simulink model "IRB120_identification"  (R2026a)
settings: Solver=ode3  StopTime=40  FixedStep=0.004
InitFcn:
  | addpath(fullfile(fileparts(get_param(bdroot, 'FileName')), 'meshes'));
values from neighbouring files (symbols this model uses):
  m = b.Mass    [extract_nominal_parameters.m]
  N = size(m.q, 1)    [build_and_simulate.m]
  s = min(t/cfg.T_ramp, 1)    [build_and_simulate.m]
  X = Tm \ getTransform(r, qm, bodies{i})    [extract_nominal_parameters.m]
undefined symbols (not defined in the file or in its folder): Y, Z
libraries: sm_lib x62, nesl_utility x31
(part 1 of 2)
settings Model: Creator=Muhammad Adel  LastModifiedBy=Muhammad Adel

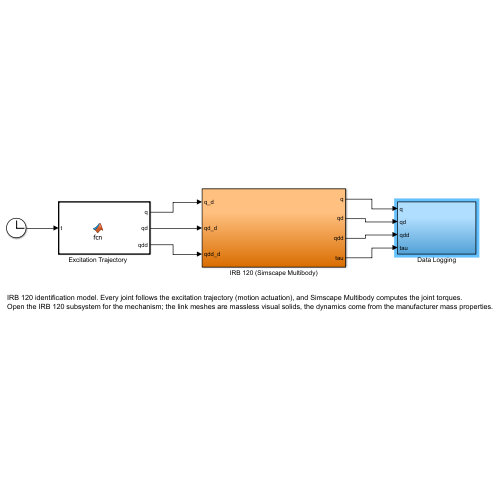
[thumbnail: Simulink's stored preview of the top-level diagram]
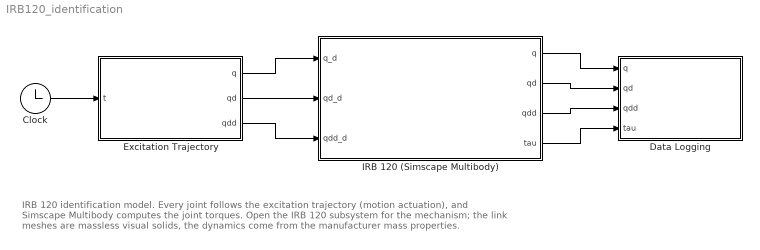
== system IRB120_identification ==
  note: IRB 120 identification model. Every joint follows the excitation trajectory (motion actuation), and Simscape Multibody computes the joint torques.
      | Open the IRB 120 subsystem for the mechanism; the link meshes are massless visual solids, the dynamics come from the manufacturer mass properties.
  Clock : Clock
  Data Logging : Subsystem
  Excitation Trajectory : MATLAB Function  TreatAsAtomicUnit=on
  IRB 120 (Simscape Multibody) : Subsystem
  wires:
  Clock/1 -> Excitation Trajectory/1(t)
  Excitation Trajectory/1(q) -> IRB 120 (Simscape Multibody)/1(q_d)
  Excitation Trajectory/2(qd) -> IRB 120 (Simscape Multibody)/2(qd_d)
  Excitation Trajectory/3(qdd) -> IRB 120 (Simscape Multibody)/3(qdd_d)
  IRB 120 (Simscape Multibody)/1(q) -> Data Logging/1(q)
  IRB 120 (Simscape Multibody)/2(qd) -> Data Logging/2(qd)
  IRB 120 (Simscape Multibody)/3(qdd) -> Data Logging/3(qdd)
  IRB 120 (Simscape Multibody)/4(tau) -> Data Logging/4(tau)

== system IRB120_identification/Data Logging ==
  q : Inport
  qd : Inport  Port=2
  qdd : Inport  Port=3
  tau : Inport  Port=4
  Log_q : ToWorkspace  VariableName=m_q  SampleTime=0.004
  Log_qd : ToWorkspace  VariableName=m_qd  SampleTime=0.004
  Log_qdd : ToWorkspace  VariableName=m_qdd  SampleTime=0.004
  Log_tau : ToWorkspace  VariableName=m_tau  SampleTime=0.004
  wires:
  qd/1 -> Log_qd/1
  q/1 -> Log_q/1
  qdd/1 -> Log_qdd/1
  tau/1 -> Log_tau/1

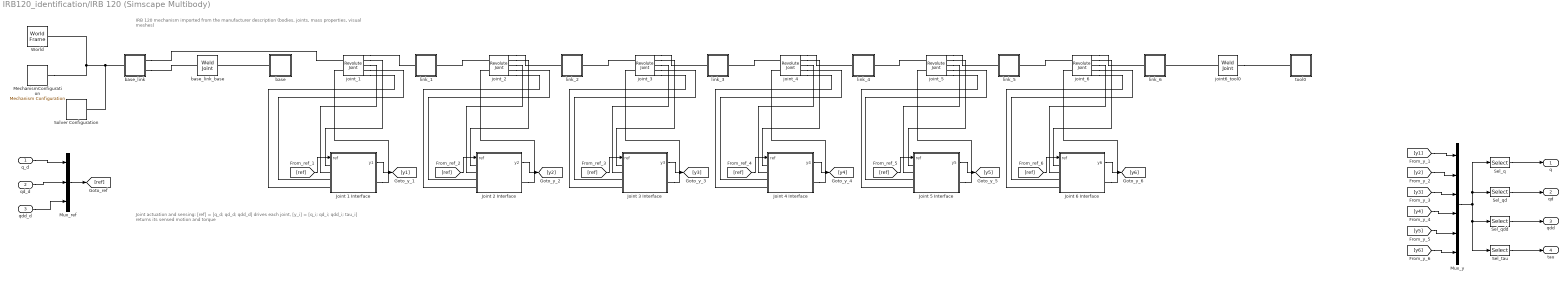
== system IRB120_identification/IRB 120 (Simscape Multibody) ==
  note: IRB 120 mechanism imported from the manufacturer description (bodies, joints, mass properties, visual meshes)
  note: Joint actuation and sensing: [ref] = [q_d; qd_d; qdd_d] drives each joint, [y_i] = [q_i; qd_i; qdd_i; tau_i] returns its sensed motion and torque
  q_d : Inport
  qd_d : Inport  Port=2
  qdd_d : Inport  Port=3
  Joint 1 Interface : Subsystem
  Joint 2 Interface : Subsystem
  Joint 3 Interface : Subsystem
  Joint 4 Interface : Subsystem
  Joint 5 Interface : Subsystem
  Joint 6 Interface : Subsystem
  MechanismConfiguration : sm_lib/Utilities/Mechanism Configuration  UniformGravity=Constant  GravityVector=[0, 0, -9.81]  GravityVectorUnits=m/s^2  LinearizationDelta=0.001  JointModeTransitionNonlinearIterations=2
  Mux_ref : Mux  Inputs=3
  Mux_y : Mux  Inputs=6
  Sel_q : Selector  InputPortWidth=24  IndexOptions=Index vector (dialog)  Indices=1:4:24  OutputSizes=1
  Sel_qd : Selector  InputPortWidth=24  IndexOptions=Index vector (dialog)  Indices=2:4:24  OutputSizes=1
  Sel_qdd : Selector  InputPortWidth=24  IndexOptions=Index vector (dialog)  Indices=3:4:24  OutputSizes=1
  Sel_tau : Selector  InputPortWidth=24  IndexOptions=Index vector (dialog)  Indices=4:4:24  OutputSizes=1
  Solver Configuration : nesl_utility/Solver Configuration  PhysicalDomain=network_engine_domain  SubClassName=solver  LeftPortType=input  RightPortType=generic  Tones=[]  Harmonics=[]  SimulateNoise=off  Profile=off  UseLocalSampling=off  EnableSwitchedLinearOptims=on  FrequencyDomain=off  UseCCode=off  RelTol=0.001  AbsTol=0.001  MinStep=1e-09  ToWorkspace=off  RevertToSquareIcSolve=off  NumHomotopyIterations=100  PhasorMode=off  PhasorModeNumHarmonics=1  ConsistencySolver=NEWTON_XTOL_AFTER_FTOL  CanonicalOrdering=CANONICAL  OptimizeIntermediates=OPTIMIZED  IndexReductionMethod=DerivativeReplacement  DoDC=off  ResidualTolerance=1e-09  ConsistencyTolSource=GLOBAL  ConsistencyAbsTol=0.001  ConsistencyRelTol=0.001  ConsistencyTolFactor=0.001  UseLocalSolver=off  LocalSolverChoice=NE_BACKWARD_EULER_ADVANCER  ResolveIndetEquations=on  FunctionEvalNumThread=1  LocalSolverSampleTime=0.001  DoFixedCost=off  MaxNonlinIter=3  MaxModeIter=2  ComputeImpulses=off  ImpulseIterations=2  LinearAlgebra=auto  LinearAlgebraNumThread=0  EquationFormulation=NE_TIME_EF  DelaysMemoryBudget=1024  AutomaticFiltering=on  FilteringTimeConstant=0.001  PartitionStorageMethod=AS_NEEDED  PartitionMemoryBudget=1024  PartitionMethod=ROBUST  MultibodyUseLocalSolver=off  MultibodyLocalSolverChoice=ODE1  MultibodyLocalSolverSampleTime=0.001
  World : sm_lib/Frames and Transforms/World Frame
  base : Subsystem
  base_link : Subsystem
  base_link_base : sm_lib/Joints/Weld Joint  JointMode=Normal  CompositeWrenchDir=FollowerOnBase  CompositeWrenchFrame=BaseFrame  SenseConstraintForce=off  SenseConstraintTorque=off  SenseTotalForce=off  SenseTotalTorque=off
  joint6_tool0 : sm_lib/Joints/Weld Joint  JointMode=Normal  CompositeWrenchDir=FollowerOnBase  CompositeWrenchFrame=BaseFrame  SenseConstraintForce=off  SenseConstraintTorque=off  SenseTotalForce=off  SenseTotalTorque=off
  joint_1 : sm_lib/Joints/Revolute Joint  JointMode=Normal  CompositeWrenchDir=FollowerOnBase  CompositeWrenchFrame=BaseFrame  SenseConstraintForce=off  SenseConstraintTorque=off  SenseTotalForce=off  SenseTotalTorque=off  PositionTargetSpecify=on  PositionTargetPriority=High  PositionTargetValue=0  PositionTargetValueUnits=rad  VelocityTargetSpecify=off  VelocityTargetPriority=High  VelocityTargetValue=0  VelocityTargetValueUnits=deg/s  EquilibriumPosition=0  EquilibriumPositionUnits=deg  SpringStiffness=0  SpringStiffnessUnits=N*m/deg  DampingCoefficient=0  DampingCoefficientUnits=kg*m^2/(rad*s)  LowerLimitSpecify=off  LowerLimitBound=-2.87979  LowerLimitBoundUnits=rad  LowerLimitStiffness=1e4  LowerLimitStiffnessUnits=N*m/deg  LowerLimitDamping=10  LowerLimitDampingUnits=N*m/(deg/s)  LowerLimitTransitionRegionWidth=0.1  LowerLimitTransitionRegionWidthUnits=deg  UpperLimitSpecify=off  UpperLimitBound=2.87979  UpperLimitBoundUnits=rad  UpperLimitStiffness=1e4  UpperLimitStiffnessUnits=N*m/deg  UpperLimitDamping=10  UpperLimitDampingUnits=N*m/(deg/s)  UpperLimitTransitionRegionWidth=0.1  UpperLimitTransitionRegionWidthUnits=deg  TorqueActuationMode=ComputedTorque  MotionActuationMode=InputMotion  SensePosition=on  SenseVelocity=on  SenseAcceleration=on  SenseTorqueForce=on  SenseLowerLimitTorqueForce=off  SenseUpperLimitTorqueForce=off
  joint_2 : sm_lib/Joints/Revolute Joint  JointMode=Normal  CompositeWrenchDir=FollowerOnBase  CompositeWrenchFrame=BaseFrame  SenseConstraintForce=off  SenseConstraintTorque=off  SenseTotalForce=off  SenseTotalTorque=off  PositionTargetSpecify=on  PositionTargetPriority=High  PositionTargetValue=0  PositionTargetValueUnits=rad  VelocityTargetSpecify=off  VelocityTargetPriority=High  VelocityTargetValue=0  VelocityTargetValueUnits=deg/s  EquilibriumPosition=0  EquilibriumPositionUnits=deg  SpringStiffness=0  SpringStiffnessUnits=N*m/deg  DampingCoefficient=0  DampingCoefficientUnits=kg*m^2/(rad*s)  LowerLimitSpecify=off  LowerLimitBound=-1.91986  LowerLimitBoundUnits=rad  LowerLimitStiffness=1e4  LowerLimitStiffnessUnits=N*m/deg  LowerLimitDamping=10  LowerLimitDampingUnits=N*m/(deg/s)  LowerLimitTransitionRegionWidth=0.1  LowerLimitTransitionRegionWidthUnits=deg  UpperLimitSpecify=off  UpperLimitBound=1.91986  UpperLimitBoundUnits=rad  UpperLimitStiffness=1e4  UpperLimitStiffnessUnits=N*m/deg  UpperLimitDamping=10  UpperLimitDampingUnits=N*m/(deg/s)  UpperLimitTransitionRegionWidth=0.1  UpperLimitTransitionRegionWidthUnits=deg  TorqueActuationMode=ComputedTorque  MotionActuationMode=InputMotion  SensePosition=on  SenseVelocity=on  SenseAcceleration=on  SenseTorqueForce=on  SenseLowerLimitTorqueForce=off  SenseUpperLimitTorqueForce=off
  joint_3 : sm_lib/Joints/Revolute Joint  JointMode=Normal  CompositeWrenchDir=FollowerOnBase  CompositeWrenchFrame=BaseFrame  SenseConstraintForce=off  SenseConstraintTorque=off  SenseTotalForce=off  SenseTotalTorque=off  PositionTargetSpecify=on  PositionTargetPriority=High  PositionTargetValue=0  PositionTargetValueUnits=rad  VelocityTargetSpecify=off  VelocityTargetPriority=High  VelocityTargetValue=0  VelocityTargetValueUnits=deg/s  EquilibriumPosition=0  EquilibriumPositionUnits=deg  SpringStiffness=0  SpringStiffnessUnits=N*m/deg  DampingCoefficient=0  DampingCoefficientUnits=kg*m^2/(rad*s)  LowerLimitSpecify=off  LowerLimitBound=-1.91986  LowerLimitBoundUnits=rad  LowerLimitStiffness=1e4  LowerLimitStiffnessUnits=N*m/deg  LowerLimitDamping=10  LowerLimitDampingUnits=N*m/(deg/s)  LowerLimitTransitionRegionWidth=0.1  LowerLimitTransitionRegionWidthUnits=deg  UpperLimitSpecify=off  UpperLimitBound=1.22173  UpperLimitBoundUnits=rad  UpperLimitStiffness=1e4  UpperLimitStiffnessUnits=N*m/deg  UpperLimitDamping=10  UpperLimitDampingUnits=N*m/(deg/s)  UpperLimitTransitionRegionWidth=0.1  UpperLimitTransitionRegionWidthUnits=deg  TorqueActuationMode=ComputedTorque  MotionActuationMode=InputMotion  SensePosition=on  SenseVelocity=on  SenseAcceleration=on  SenseTorqueForce=on  SenseLowerLimitTorqueForce=off  SenseUpperLimitTorqueForce=off
  joint_4 : sm_lib/Joints/Revolute Joint  JointMode=Normal  CompositeWrenchDir=FollowerOnBase  CompositeWrenchFrame=BaseFrame  SenseConstraintForce=off  SenseConstraintTorque=off  SenseTotalForce=off  SenseTotalTorque=off  PositionTargetSpecify=on  PositionTargetPriority=High  PositionTargetValue=0  PositionTargetValueUnits=rad  VelocityTargetSpecify=off  VelocityTargetPriority=High  VelocityTargetValue=0  VelocityTargetValueUnits=deg/s  EquilibriumPosition=0  EquilibriumPositionUnits=deg  SpringStiffness=0  SpringStiffnessUnits=N*m/deg  DampingCoefficient=0  DampingCoefficientUnits=kg*m^2/(rad*s)  LowerLimitSpecify=off  LowerLimitBound=-2.79253  LowerLimitBoundUnits=rad  LowerLimitStiffness=1e4  LowerLimitStiffnessUnits=N*m/deg  LowerLimitDamping=10  LowerLimitDampingUnits=N*m/(deg/s)  LowerLimitTransitionRegionWidth=0.1  LowerLimitTransitionRegionWidthUnits=deg  UpperLimitSpecify=off  UpperLimitBound=2.79253  UpperLimitBoundUnits=rad  UpperLimitStiffness=1e4  UpperLimitStiffnessUnits=N*m/deg  UpperLimitDamping=10  UpperLimitDampingUnits=N*m/(deg/s)  UpperLimitTransitionRegionWidth=0.1  UpperLimitTransitionRegionWidthUnits=deg  TorqueActuationMode=ComputedTorque  MotionActuationMode=InputMotion  SensePosition=on  SenseVelocity=on  SenseAcceleration=on  SenseTorqueForce=on  SenseLowerLimitTorqueForce=off  SenseUpperLimitTorqueForce=off
  joint_5 : sm_lib/Joints/Revolute Joint  JointMode=Normal  CompositeWrenchDir=FollowerOnBase  CompositeWrenchFrame=BaseFrame  SenseConstraintForce=off  SenseConstraintTorque=off  SenseTotalForce=off  SenseTotalTorque=off  PositionTargetSpecify=on  PositionTargetPriority=High  PositionTargetValue=0  PositionTargetValueUnits=rad  VelocityTargetSpecify=off  VelocityTargetPriority=High  VelocityTargetValue=0  VelocityTargetValueUnits=deg/s  EquilibriumPosition=0  EquilibriumPositionUnits=deg  SpringStiffness=0  SpringStiffnessUnits=N*m/deg  DampingCoefficient=0  DampingCoefficientUnits=kg*m^2/(rad*s)  LowerLimitSpecify=off  LowerLimitBound=-2.094395  LowerLimitBoundUnits=rad  LowerLimitStiffness=1e4  LowerLimitStiffnessUnits=N*m/deg  LowerLimitDamping=10  LowerLimitDampingUnits=N*m/(deg/s)  LowerLimitTransitionRegionWidth=0.1  LowerLimitTransitionRegionWidthUnits=deg  UpperLimitSpecify=off  UpperLimitBound=2.094395  UpperLimitBoundUnits=rad  UpperLimitStiffness=1e4  UpperLimitStiffnessUnits=N*m/deg  UpperLimitDamping=10  UpperLimitDampingUnits=N*m/(deg/s)  UpperLimitTransitionRegionWidth=0.1  UpperLimitTransitionRegionWidthUnits=deg  TorqueActuationMode=ComputedTorque  MotionActuationMode=InputMotion  SensePosition=on  SenseVelocity=on  SenseAcceleration=on  SenseTorqueForce=on  SenseLowerLimitTorqueForce=off  SenseUpperLimitTorqueForce=off
  joint_6 : sm_lib/Joints/Revolute Joint  JointMode=Normal  CompositeWrenchDir=FollowerOnBase  CompositeWrenchFrame=BaseFrame  SenseConstraintForce=off  SenseConstraintTorque=off  SenseTotalForce=off  SenseTotalTorque=off  PositionTargetSpecify=on  PositionTargetPriority=High  PositionTargetValue=0  PositionTargetValueUnits=rad  VelocityTargetSpecify=off  VelocityTargetPriority=High  VelocityTargetValue=0  VelocityTargetValueUnits=deg/s  EquilibriumPosition=0  EquilibriumPositionUnits=deg  SpringStiffness=0  SpringStiffnessUnits=N*m/deg  DampingCoefficient=0  DampingCoefficientUnits=kg*m^2/(rad*s)  LowerLimitSpecify=off  LowerLimitBound=-6.98132  LowerLimitBoundUnits=rad  LowerLimitStiffness=1e4  LowerLimitStiffnessUnits=N*m/deg  LowerLimitDamping=10  LowerLimitDampingUnits=N*m/(deg/s)  LowerLimitTransitionRegionWidth=0.1  LowerLimitTransitionRegionWidthUnits=deg  UpperLimitSpecify=off  UpperLimitBound=6.98132  UpperLimitBoundUnits=rad  UpperLimitStiffness=1e4  UpperLimitStiffnessUnits=N*m/deg  UpperLimitDamping=10  UpperLimitDampingUnits=N*m/(deg/s)  UpperLimitTransitionRegionWidth=0.1  UpperLimitTransitionRegionWidthUnits=deg  TorqueActuationMode=ComputedTorque  MotionActuationMode=InputMotion  SensePosition=on  SenseVelocity=on  SenseAcceleration=on  SenseTorqueForce=on  SenseLowerLimitTorqueForce=off  SenseUpperLimitTorqueForce=off
  link_1 : Subsystem
  link_2 : Subsystem
  link_3 : Subsystem
  link_4 : Subsystem
  link_5 : Subsystem
  link_6 : Subsystem
  tool0 : Subsystem
  q : Outport
  qd : Outport  Port=2
  qdd : Outport  Port=3
  tau : Outport  Port=4
  wires:
  Joint 5 Interface/1(y5) -> [y5]
  Mux_ref/1 -> [ref]
  [ref] -> Joint 4 Interface/1(ref)
  Joint 4 Interface/1(y4) -> [y4]
  [ref] -> Joint 6 Interface/1(ref)
  Joint 6 Interface/1(y6) -> [y6]
  Mux_y/1 -> Sel_qdd/1, Sel_tau/1, Sel_q/1, Sel_qd/1
  Joint 3 Interface/1(y3) -> [y3]
  [ref] -> Joint 1 Interface/1(ref)
  Joint 1 Interface/1(y1) -> [y1]
  Sel_q/1 -> q/1
  Joint 2 Interface/1(y2) -> [y2]
  [ref] -> Joint 2 Interface/1(ref)
  [y6] -> Mux_y/6
  [ref] -> Joint 3 Interface/1(ref)
  [y2] -> Mux_y/2
  [ref] -> Joint 5 Interface/1(ref)
  [y1] -> Mux_y/1
  [y3] -> Mux_y/3
  [y4] -> Mux_y/4
  [y5] -> Mux_y/5
  q_d/1 -> Mux_ref/1
  qdd_d/1 -> Mux_ref/3
  qd_d/1 -> Mux_ref/2
  Sel_qdd/1 -> qdd/1
  Sel_tau/1 -> tau/1
  Sel_qd/1 -> qd/1
  connections:
  joint_4/RConn5 -- Joint 4 Interface/LConn4
  joint_3/RConn4 -- Joint 3 Interface/LConn3
  joint_5/RConn2 -- Joint 5 Interface/LConn1
  joint_3/LConn1 -- link_2/RConn1
  joint_3/RConn2 -- Joint 3 Interface/LConn1
  joint_6/RConn5 -- Joint 6 Interface/LConn4
  joint_4/LConn1 -- link_3/RConn1
  Joint 6 Interface/RConn1 -- joint_6/LConn2
  joint_5/RConn5 -- Joint 5 Interface/LConn4
  joint_5/RConn1 -- link_5/LConn1
  joint_3/RConn3 -- Joint 3 Interface/LConn2
  joint_4/RConn4 -- Joint 4 Interface/LConn3
  joint6_tool0/LConn1 -- link_6/RConn1
  joint_4/RConn2 -- Joint 4 Interface/LConn1
  joint_1/RConn2 -- Joint 1 Interface/LConn1
  joint_4/RConn3 -- Joint 4 Interface/LConn2
  joint_1/RConn5 -- Joint 1 Interface/LConn4
  joint6_tool0/RConn1 -- tool0/LConn1
  base_link/RConn1 -- joint_1/LConn1
  Joint 4 Interface/RConn1 -- joint_4/LConn2
  World/RConn1 -- base_link/LConn1 -- Solver Configuration/RConn1 -- MechanismConfiguration/RConn1
  joint_1/RConn3 -- Joint 1 Interface/LConn2
  Joint 2 Interface/RConn1 -- joint_2/LConn2
  joint_3/RConn5 -- Joint 3 Interface/LConn4
  joint_2/RConn1 -- link_2/LConn1
  joint_5/RConn3 -- Joint 5 Interface/LConn2
  joint_2/LConn1 -- link_1/RConn1
  joint_6/LConn1 -- link_5/RConn1
  joint_6/RConn4 -- Joint 6 Interface/LConn3
  joint_2/RConn2 -- Joint 2 Interface/LConn1
  base_link/RConn2 -- base_link_base/LConn1
  joint_6/RConn1 -- link_6/LConn1
  Joint 5 Interface/RConn1 -- joint_5/LConn2
  Joint 3 Interface/RConn1 -- joint_3/LConn2
  joint_1/RConn1 -- link_1/LConn1
  joint_4/RConn1 -- link_4/LConn1
  joint_5/LConn1 -- link_4/RConn1
  base/LConn1 -- base_link_base/RConn1
  joint_3/RConn1 -- link_3/LConn1
  joint_1/RConn4 -- Joint 1 Interface/LConn3
  Joint 1 Interface/RConn1 -- joint_1/LConn2
  joint_2/RConn4 -- Joint 2 Interface/LConn3
  joint_2/RConn3 -- Joint 2 Interface/LConn2
  joint_2/RConn5 -- Joint 2 Interface/LConn4
  joint_5/RConn4 -- Joint 5 Interface/LConn3
  joint_6/RConn2 -- Joint 6 Interface/LConn1
  joint_6/RConn3 -- Joint 6 Interface/LConn2

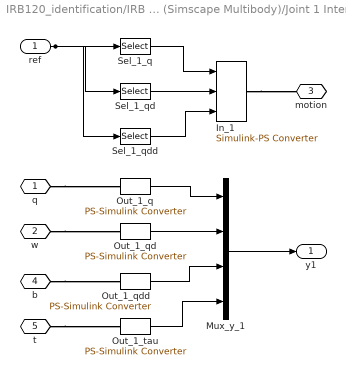
== system IRB120_identification/IRB 120 (Simscape Multibody)/Joint 1 Interface ==
  ref : Inport
  In_1 : nesl_utility/Simulink-PS Converter  PhysicalDomain=network_engine_domain  SubClassName=ps_input  LeftPortType=input  RightPortType=output  PseudoPeriodic=off  Frequencies=[]  NoiseDistribution=none  NoiseParameters=[]  Unit=rad  AffineConversion=off  FilteringAndDerivatives=provide  SimscapeFilterOrder=1  InputFilterTimeConstant=0.001  UdotUserProvided=2
  Mux_y_1 : Mux
  Out_1_q : nesl_utility/PS-Simulink Converter  PhysicalDomain=network_engine_domain  SubClassName=ps_output  LeftPortType=input  RightPortType=output  PseudoPeriodic=off  Frequencies=[]  VectorFormat=inherit  Unit=rad  AffineConversion=off
  Out_1_qd : nesl_utility/PS-Simulink Converter  PhysicalDomain=network_engine_domain  SubClassName=ps_output  LeftPortType=input  RightPortType=output  PseudoPeriodic=off  Frequencies=[]  VectorFormat=inherit  Unit=rad/s  AffineConversion=off
  Out_1_qdd : nesl_utility/PS-Simulink Converter  PhysicalDomain=network_engine_domain  SubClassName=ps_output  LeftPortType=input  RightPortType=output  PseudoPeriodic=off  Frequencies=[]  VectorFormat=inherit  Unit=rad/s^2  AffineConversion=off
  Out_1_tau : nesl_utility/PS-Simulink Converter  PhysicalDomain=network_engine_domain  SubClassName=ps_output  LeftPortType=input  RightPortType=output  PseudoPeriodic=off  Frequencies=[]  VectorFormat=inherit  Unit=N*m  AffineConversion=off
  Sel_1_q : Selector  InputPortWidth=18  IndexOptions=Index vector (dialog)  Indices=1  OutputSizes=1
  Sel_1_qd : Selector  InputPortWidth=18  IndexOptions=Index vector (dialog)  Indices=7  OutputSizes=1
  Sel_1_qdd : Selector  InputPortWidth=18  IndexOptions=Index vector (dialog)  Indices=13  OutputSizes=1
  q : PMIOPort  Side=Left
  w : PMIOPort  Port=2  Side=Left
  motion : PMIOPort  Port=3  Side=Right
  b : PMIOPort  Port=4  Side=Left
  t : PMIOPort  Port=5  Side=Left
  y1 : Outport
  wires:
  ref/1 -> Sel_1_q/1, Sel_1_qdd/1, Sel_1_qd/1
  Sel_1_q/1 -> In_1/1
  Sel_1_qdd/1 -> In_1/3
  Sel_1_qd/1 -> In_1/2
  Mux_y_1/1 -> y1/1
  Out_1_q/1 -> Mux_y_1/1
  Out_1_qd/1 -> Mux_y_1/2
  Out_1_qdd/1 -> Mux_y_1/3
  Out_1_tau/1 -> Mux_y_1/4
  connections:
  t/RConn1 -- Out_1_tau/LConn1
  b/RConn1 -- Out_1_qdd/LConn1
  w/RConn1 -- Out_1_qd/LConn1
  q/RConn1 -- Out_1_q/LConn1
  In_1/RConn1 -- motion/RConn1

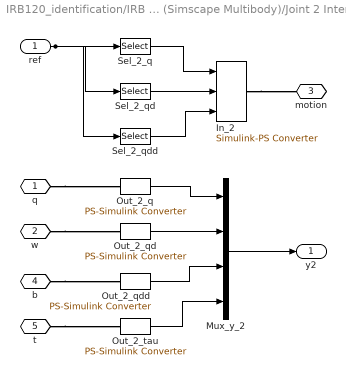
== system IRB120_identification/IRB 120 (Simscape Multibody)/Joint 2 Interface ==
  ref : Inport
  In_2 : nesl_utility/Simulink-PS Converter  PhysicalDomain=network_engine_domain  SubClassName=ps_input  LeftPortType=input  RightPortType=output  PseudoPeriodic=off  Frequencies=[]  NoiseDistribution=none  NoiseParameters=[]  Unit=rad  AffineConversion=off  FilteringAndDerivatives=provide  SimscapeFilterOrder=1  InputFilterTimeConstant=0.001  UdotUserProvided=2
  Mux_y_2 : Mux
  Out_2_q : nesl_utility/PS-Simulink Converter  PhysicalDomain=network_engine_domain  SubClassName=ps_output  LeftPortType=input  RightPortType=output  PseudoPeriodic=off  Frequencies=[]  VectorFormat=inherit  Unit=rad  AffineConversion=off
  Out_2_qd : nesl_utility/PS-Simulink Converter  PhysicalDomain=network_engine_domain  SubClassName=ps_output  LeftPortType=input  RightPortType=output  PseudoPeriodic=off  Frequencies=[]  VectorFormat=inherit  Unit=rad/s  AffineConversion=off
  Out_2_qdd : nesl_utility/PS-Simulink Converter  PhysicalDomain=network_engine_domain  SubClassName=ps_output  LeftPortType=input  RightPortType=output  PseudoPeriodic=off  Frequencies=[]  VectorFormat=inherit  Unit=rad/s^2  AffineConversion=off
  Out_2_tau : nesl_utility/PS-Simulink Converter  PhysicalDomain=network_engine_domain  SubClassName=ps_output  LeftPortType=input  RightPortType=output  PseudoPeriodic=off  Frequencies=[]  VectorFormat=inherit  Unit=N*m  AffineConversion=off
  Sel_2_q : Selector  InputPortWidth=18  IndexOptions=Index vector (dialog)  Indices=2  OutputSizes=1
  Sel_2_qd : Selector  InputPortWidth=18  IndexOptions=Index vector (dialog)  Indices=8  OutputSizes=1
  Sel_2_qdd : Selector  InputPortWidth=18  IndexOptions=Index vector (dialog)  Indices=14  OutputSizes=1
  q : PMIOPort  Side=Left
  w : PMIOPort  Port=2  Side=Left
  motion : PMIOPort  Port=3  Side=Right
  b : PMIOPort  Port=4  Side=Left
  t : PMIOPort  Port=5  Side=Left
  y2 : Outport
  wires:
  ref/1 -> Sel_2_qd/1, Sel_2_qdd/1, Sel_2_q/1
  Sel_2_q/1 -> In_2/1
  Sel_2_qdd/1 -> In_2/3
  Sel_2_qd/1 -> In_2/2
  Out_2_q/1 -> Mux_y_2/1
  Out_2_qd/1 -> Mux_y_2/2
  Out_2_qdd/1 -> Mux_y_2/3
  Out_2_tau/1 -> Mux_y_2/4
  Mux_y_2/1 -> y2/1
  connections:
  t/RConn1 -- Out_2_tau/LConn1
  q/RConn1 -- Out_2_q/LConn1
  b/RConn1 -- Out_2_qdd/LConn1
  w/RConn1 -- Out_2_qd/LConn1
  In_2/RConn1 -- motion/RConn1

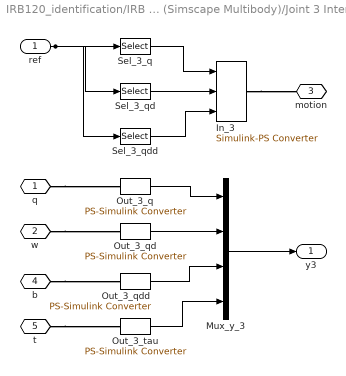
== system IRB120_identification/IRB 120 (Simscape Multibody)/Joint 3 Interface ==
  ref : Inport
  In_3 : nesl_utility/Simulink-PS Converter  PhysicalDomain=network_engine_domain  SubClassName=ps_input  LeftPortType=input  RightPortType=output  PseudoPeriodic=off  Frequencies=[]  NoiseDistribution=none  NoiseParameters=[]  Unit=rad  AffineConversion=off  FilteringAndDerivatives=provide  SimscapeFilterOrder=1  InputFilterTimeConstant=0.001  UdotUserProvided=2
  Mux_y_3 : Mux
  Out_3_q : nesl_utility/PS-Simulink Converter  PhysicalDomain=network_engine_domain  SubClassName=ps_output  LeftPortType=input  RightPortType=output  PseudoPeriodic=off  Frequencies=[]  VectorFormat=inherit  Unit=rad  AffineConversion=off
  Out_3_qd : nesl_utility/PS-Simulink Converter  PhysicalDomain=network_engine_domain  SubClassName=ps_output  LeftPortType=input  RightPortType=output  PseudoPeriodic=off  Frequencies=[]  VectorFormat=inherit  Unit=rad/s  AffineConversion=off
  Out_3_qdd : nesl_utility/PS-Simulink Converter  PhysicalDomain=network_engine_domain  SubClassName=ps_output  LeftPortType=input  RightPortType=output  PseudoPeriodic=off  Frequencies=[]  VectorFormat=inherit  Unit=rad/s^2  AffineConversion=off
  Out_3_tau : nesl_utility/PS-Simulink Converter  PhysicalDomain=network_engine_domain  SubClassName=ps_output  LeftPortType=input  RightPortType=output  PseudoPeriodic=off  Frequencies=[]  VectorFormat=inherit  Unit=N*m  AffineConversion=off
  Sel_3_q : Selector  InputPortWidth=18  IndexOptions=Index vector (dialog)  Indices=3  OutputSizes=1
  Sel_3_qd : Selector  InputPortWidth=18  IndexOptions=Index vector (dialog)  Indices=9  OutputSizes=1
  Sel_3_qdd : Selector  InputPortWidth=18  IndexOptions=Index vector (dialog)  Indices=15  OutputSizes=1
  q : PMIOPort  Side=Left
  w : PMIOPort  Port=2  Side=Left
  motion : PMIOPort  Port=3  Side=Right
  b : PMIOPort  Port=4  Side=Left
  t : PMIOPort  Port=5  Side=Left
  y3 : Outport
  wires:
  Out_3_tau/1 -> Mux_y_3/4
  ref/1 -> Sel_3_q/1, Sel_3_qd/1, Sel_3_qdd/1
  Out_3_qdd/1 -> Mux_y_3/3
  Sel_3_q/1 -> In_3/1
  Out_3_qd/1 -> Mux_y_3/2
  Sel_3_qdd/1 -> In_3/3
  Sel_3_qd/1 -> In_3/2
  Mux_y_3/1 -> y3/1
  Out_3_q/1 -> Mux_y_3/1
  connections:
  t/RConn1 -- Out_3_tau/LConn1
  q/RConn1 -- Out_3_q/LConn1
  b/RConn1 -- Out_3_qdd/LConn1
  w/RConn1 -- Out_3_qd/LConn1
  In_3/RConn1 -- motion/RConn1

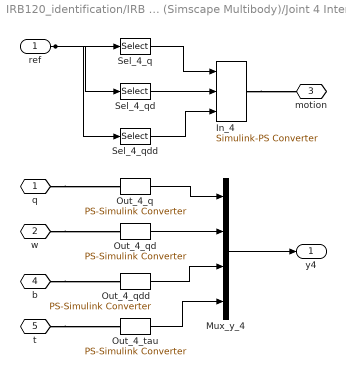
== system IRB120_identification/IRB 120 (Simscape Multibody)/Joint 4 Interface ==
  ref : Inport
  In_4 : nesl_utility/Simulink-PS Converter  PhysicalDomain=network_engine_domain  SubClassName=ps_input  LeftPortType=input  RightPortType=output  PseudoPeriodic=off  Frequencies=[]  NoiseDistribution=none  NoiseParameters=[]  Unit=rad  AffineConversion=off  FilteringAndDerivatives=provide  SimscapeFilterOrder=1  InputFilterTimeConstant=0.001  UdotUserProvided=2
  Mux_y_4 : Mux
  Out_4_q : nesl_utility/PS-Simulink Converter  PhysicalDomain=network_engine_domain  SubClassName=ps_output  LeftPortType=input  RightPortType=output  PseudoPeriodic=off  Frequencies=[]  VectorFormat=inherit  Unit=rad  AffineConversion=off
  Out_4_qd : nesl_utility/PS-Simulink Converter  PhysicalDomain=network_engine_domain  SubClassName=ps_output  LeftPortType=input  RightPortType=output  PseudoPeriodic=off  Frequencies=[]  VectorFormat=inherit  Unit=rad/s  AffineConversion=off
  Out_4_qdd : nesl_utility/PS-Simulink Converter  PhysicalDomain=network_engine_domain  SubClassName=ps_output  LeftPortType=input  RightPortType=output  PseudoPeriodic=off  Frequencies=[]  VectorFormat=inherit  Unit=rad/s^2  AffineConversion=off
  Out_4_tau : nesl_utility/PS-Simulink Converter  PhysicalDomain=network_engine_domain  SubClassName=ps_output  LeftPortType=input  RightPortType=output  PseudoPeriodic=off  Frequencies=[]  VectorFormat=inherit  Unit=N*m  AffineConversion=off
  Sel_4_q : Selector  InputPortWidth=18  IndexOptions=Index vector (dialog)  Indices=4  OutputSizes=1
  Sel_4_qd : Selector  InputPortWidth=18  IndexOptions=Index vector (dialog)  Indices=10  OutputSizes=1
  Sel_4_qdd : Selector  InputPortWidth=18  IndexOptions=Index vector (dialog)  Indices=16  OutputSizes=1
  q : PMIOPort  Side=Left
  w : PMIOPort  Port=2  Side=Left
  motion : PMIOPort  Port=3  Side=Right
  b : PMIOPort  Port=4  Side=Left
  t : PMIOPort  Port=5  Side=Left
  y4 : Outport
  wires:
  Out_4_tau/1 -> Mux_y_4/4
  ref/1 -> Sel_4_q/1, Sel_4_qd/1, Sel_4_qdd/1
  Sel_4_q/1 -> In_4/1
  Sel_4_qdd/1 -> In_4/3
  Sel_4_qd/1 -> In_4/2
  Out_4_q/1 -> Mux_y_4/1
  Out_4_qd/1 -> Mux_y_4/2
  Out_4_qdd/1 -> Mux_y_4/3
  Mux_y_4/1 -> y4/1
  connections:
  t/RConn1 -- Out_4_tau/LConn1
  q/RConn1 -- Out_4_q/LConn1
  b/RConn1 -- Out_4_qdd/LConn1
  w/RConn1 -- Out_4_qd/LConn1
  In_4/RConn1 -- motion/RConn1

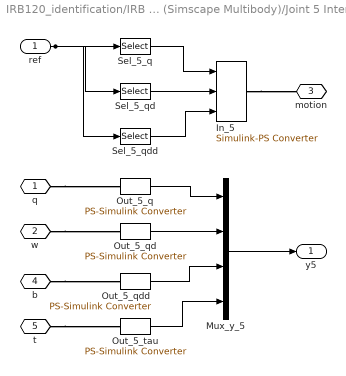
== system IRB120_identification/IRB 120 (Simscape Multibody)/Joint 5 Interface ==
  ref : Inport
  In_5 : nesl_utility/Simulink-PS Converter  PhysicalDomain=network_engine_domain  SubClassName=ps_input  LeftPortType=input  RightPortType=output  PseudoPeriodic=off  Frequencies=[]  NoiseDistribution=none  NoiseParameters=[]  Unit=rad  AffineConversion=off  FilteringAndDerivatives=provide  SimscapeFilterOrder=1  InputFilterTimeConstant=0.001  UdotUserProvided=2
  Mux_y_5 : Mux
  Out_5_q : nesl_utility/PS-Simulink Converter  PhysicalDomain=network_engine_domain  SubClassName=ps_output  LeftPortType=input  RightPortType=output  PseudoPeriodic=off  Frequencies=[]  VectorFormat=inherit  Unit=rad  AffineConversion=off
  Out_5_qd : nesl_utility/PS-Simulink Converter  PhysicalDomain=network_engine_domain  SubClassName=ps_output  LeftPortType=input  RightPortType=output  PseudoPeriodic=off  Frequencies=[]  VectorFormat=inherit  Unit=rad/s  AffineConversion=off
  Out_5_qdd : nesl_utility/PS-Simulink Converter  PhysicalDomain=network_engine_domain  SubClassName=ps_output  LeftPortType=input  RightPortType=output  PseudoPeriodic=off  Frequencies=[]  VectorFormat=inherit  Unit=rad/s^2  AffineConversion=off
  Out_5_tau : nesl_utility/PS-Simulink Converter  PhysicalDomain=network_engine_domain  SubClassName=ps_output  LeftPortType=input  RightPortType=output  PseudoPeriodic=off  Frequencies=[]  VectorFormat=inherit  Unit=N*m  AffineConversion=off
  Sel_5_q : Selector  InputPortWidth=18  IndexOptions=Index vector (dialog)  Indices=5  OutputSizes=1
  Sel_5_qd : Selector  InputPortWidth=18  IndexOptions=Index vector (dialog)  Indices=11  OutputSizes=1
  Sel_5_qdd : Selector  InputPortWidth=18  IndexOptions=Index vector (dialog)  Indices=17  OutputSizes=1
  q : PMIOPort  Side=Left
  w : PMIOPort  Port=2  Side=Left
  motion : PMIOPort  Port=3  Side=Right
  b : PMIOPort  Port=4  Side=Left
  t : PMIOPort  Port=5  Side=Left
  y5 : Outport
  wires:
  Out_5_tau/1 -> Mux_y_5/4
  ref/1 -> Sel_5_qd/1, Sel_5_q/1, Sel_5_qdd/1
  Sel_5_q/1 -> In_5/1
  Sel_5_qdd/1 -> In_5/3
  Sel_5_qd/1 -> In_5/2
  Mux_y_5/1 -> y5/1
  Out_5_q/1 -> Mux_y_5/1
  Out_5_qd/1 -> Mux_y_5/2
  Out_5_qdd/1 -> Mux_y_5/3
  connections:
  q/RConn1 -- Out_5_q/LConn1
  w/RConn1 -- Out_5_qd/LConn1
  b/RConn1 -- Out_5_qdd/LConn1
  t/RConn1 -- Out_5_tau/LConn1
  In_5/RConn1 -- motion/RConn1

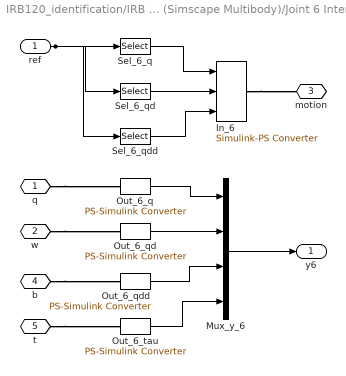
== system IRB120_identification/IRB 120 (Simscape Multibody)/Joint 6 Interface ==
  ref : Inport
  In_6 : nesl_utility/Simulink-PS Converter  PhysicalDomain=network_engine_domain  SubClassName=ps_input  LeftPortType=input  RightPortType=output  PseudoPeriodic=off  Frequencies=[]  NoiseDistribution=none  NoiseParameters=[]  Unit=rad  AffineConversion=off  FilteringAndDerivatives=provide  SimscapeFilterOrder=1  InputFilterTimeConstant=0.001  UdotUserProvided=2
  Mux_y_6 : Mux
  Out_6_q : nesl_utility/PS-Simulink Converter  PhysicalDomain=network_engine_domain  SubClassName=ps_output  LeftPortType=input  RightPortType=output  PseudoPeriodic=off  Frequencies=[]  VectorFormat=inherit  Unit=rad  AffineConversion=off
  Out_6_qd : nesl_utility/PS-Simulink Converter  PhysicalDomain=network_engine_domain  SubClassName=ps_output  LeftPortType=input  RightPortType=output  PseudoPeriodic=off  Frequencies=[]  VectorFormat=inherit  Unit=rad/s  AffineConversion=off
  Out_6_qdd : nesl_utility/PS-Simulink Converter  PhysicalDomain=network_engine_domain  SubClassName=ps_output  LeftPortType=input  RightPortType=output  PseudoPeriodic=off  Frequencies=[]  VectorFormat=inherit  Unit=rad/s^2  AffineConversion=off
  Out_6_tau : nesl_utility/PS-Simulink Converter  PhysicalDomain=network_engine_domain  SubClassName=ps_output  LeftPortType=input  RightPortType=output  PseudoPeriodic=off  Frequencies=[]  VectorFormat=inherit  Unit=N*m  AffineConversion=off
  Sel_6_q : Selector  InputPortWidth=18  IndexOptions=Index vector (dialog)  Indices=6  OutputSizes=1
  Sel_6_qd : Selector  InputPortWidth=18  IndexOptions=Index vector (dialog)  Indices=12  OutputSizes=1
  Sel_6_qdd : Selector  InputPortWidth=18  IndexOptions=Index vector (dialog)  Indices=18  OutputSizes=1
  q : PMIOPort  Side=Left
  w : PMIOPort  Port=2  Side=Left
  motion : PMIOPort  Port=3  Side=Right
  b : PMIOPort  Port=4  Side=Left
  t : PMIOPort  Port=5  Side=Left
  y6 : Outport
  wires:
  Out_6_tau/1 -> Mux_y_6/4
  ref/1 -> Sel_6_qd/1, Sel_6_qdd/1, Sel_6_q/1
  Sel_6_q/1 -> In_6/1
  Sel_6_qd/1 -> In_6/2
  Out_6_qd/1 -> Mux_y_6/2
  Sel_6_qdd/1 -> In_6/3
  Mux_y_6/1 -> y6/1
  Out_6_q/1 -> Mux_y_6/1
  Out_6_qdd/1 -> Mux_y_6/3
  connections:
  t/RConn1 -- Out_6_tau/LConn1
  q/RConn1 -- Out_6_q/LConn1
  b/RConn1 -- Out_6_qdd/LConn1
  w/RConn1 -- Out_6_qd/LConn1
  In_6/RConn1 -- motion/RConn1

== system IRB120_identification/IRB 120 (Simscape Multibody)/base ==
  Inertia : sm_lib/Body Elements/Inertia  InertiaType=Custom  Mass=0  MassUnits=kg  CenterOfMass=[0, 0, 0]  CenterOfMassUnits=m  MomentsOfInertia=[0, 0, 0]  MomentsOfInertiaUnits=kg*m^2  ProductsOfInertia=[0, 0, 0]  ProductsOfInertiaUnits=kg*m^2  GraphicType=None  MarkerShape=Inertia  MarkerSize=20  GraphicVisPropType=SimpleVisualProperties  GraphicDiffuseColor=[0.5 0.5 0.5]  GraphicOpacity=1  GraphicSpecularColor=[0.5 0.5 0.5 1.0]  GraphicAmbientColor=[0.15 0.15 0.15 1.0]  GraphicEmissiveColor=[0.0 0.0 0.0 1.0]  GraphicShininess=75
  InertiaOriginTransform : sm_lib/Frames and Transforms/Rigid Transform  RotationMethod=RotationSequence  FollAlignAxisA=+X  BaseAlignAxisA=+Y  FollAlignAxisB=+Y  BaseAlignAxisB=+Z  RotationStandardAxis=+Z  RotationAngle=0  RotationAngleUnits=deg  RotationArbitraryAxis=[0 0 1]  RotationSequenceAxes=BaseAxes  RotationSequence=XYZ  RotationSequenceAngles=[0, 0, 0]  RotationSequenceAnglesUnits=rad  RotationMatrix=[1 0 0;0 1 0;0 0 1]  Quaternion=[1 0 0 0]  TranslationMethod=Cartesian  TranslationCartesianOffset=[0, 0, 0]  TranslationCartesianOffsetUnits=m  TranslationStandardAxis=+Z  TranslationStandardOffset=0  TranslationStandardOffsetUnits=m  TranslationROffset=0  TranslationROffsetUnits=m  TranslationThetaOffset=0  TranslationThetaOffsetUnits=deg  TranslationZOffset=0  TranslationZOffsetUnits=m
  ReferenceFrame : sm_lib/Frames and Transforms/Reference Frame
  F : PMIOPort  Side=Left
  connections:
  Inertia/RConn1 -- InertiaOriginTransform/RConn1
  ReferenceFrame/RConn1 -- InertiaOriginTransform/LConn1 -- F/RConn1

== system IRB120_identification/IRB 120 (Simscape Multibody)/base_link ==
  ReferenceFrame : sm_lib/Frames and Transforms/Reference Frame
  Visual : sm_lib/Body Elements/File Solid  ExtGeomFileName=IRB120_base_link.stl  UnitType=Custom  ExtGeomFileUnits=m  StepReaderType=HEX  ExportConvexHullGeometry=off  InertiaType=PointMass  BasedOnType=DensityFromFile  Density=1000  DensityUnits=kg/m^3  Mass=0  MassUnits=kg  CenterOfMass=[0 0 0]  CenterOfMassUnits=m  MomentsOfInertia=[1 1 1]  MomentsOfInertiaUnits=kg*m^2  ProductsOfInertia=[0 0 0]  ProductsOfInertiaUnits=kg*m^2  GraphicType=FromGeometry  MarkerShape=Sphere  MarkerSize=10  GraphicVisPropType=SimpleVisualProperties  GraphicDiffuseColor=[0.24 0.55 0.37]  GraphicOpacity=1  GraphicSpecularColor=[0.5 0.5 0.5 1.0]  GraphicAmbientColor=[0.15 0.15 0.15 1.0]  GraphicEmissiveColor=[0.0 0.0 0.0 1.0]  GraphicShininess=75  DoExposeReferenceFrame=on  SerializedFrames=<Frames/>
  base_link_base_OriginTransform : sm_lib/Frames and Transforms/Rigid Transform  RotationMethod=RotationSequence  FollAlignAxisA=+X  BaseAlignAxisA=+Y  FollAlignAxisB=+Y  BaseAlignAxisB=+Z  RotationStandardAxis=+Z  RotationAngle=0  RotationAngleUnits=deg  RotationArbitraryAxis=[0 0 1]  RotationSequenceAxes=BaseAxes  RotationSequence=XYZ  RotationSequenceAngles=[0, -0, 0]  RotationSequenceAnglesUnits=rad  RotationMatrix=[1 0 0;0 1 0;0 0 1]  Quaternion=[1 0 0 0]  TranslationMethod=Cartesian  TranslationCartesianOffset=[0, 0, 0]  TranslationCartesianOffsetUnits=m  TranslationStandardAxis=+Z  TranslationStandardOffset=0  TranslationStandardOffsetUnits=m  TranslationROffset=0  TranslationROffsetUnits=m  TranslationThetaOffset=0  TranslationThetaOffsetUnits=deg  TranslationZOffset=0  TranslationZOffsetUnits=m
  joint_1_AxisTransform : sm_lib/Frames and Transforms/Rigid Transform  RotationMethod=ArbitraryAxis  FollAlignAxisA=+X  BaseAlignAxisA=+Y  FollAlignAxisB=+Y  BaseAlignAxisB=+Z  RotationStandardAxis=+Z  RotationAngle=0  RotationAngleUnits=rad  RotationArbitraryAxis=[1, 0, 0]  RotationSequenceAxes=FollowerAxes  RotationSequence=XYX  RotationSequenceAngles=[0 0 0]  RotationSequenceAnglesUnits=deg  RotationMatrix=[1 0 0;0 1 0;0 0 1]  Quaternion=[1 0 0 0]  TranslationMethod=Cartesian  TranslationCartesianOffset=[0, 0, 0]  TranslationCartesianOffsetUnits=m  TranslationStandardAxis=+Z  TranslationStandardOffset=0  TranslationStandardOffsetUnits=m  TranslationROffset=0  TranslationROffsetUnits=m  TranslationThetaOffset=0  TranslationThetaOffsetUnits=deg  TranslationZOffset=0  TranslationZOffsetUnits=m
  joint_1_OriginTransform : sm_lib/Frames and Transforms/Rigid Transform  RotationMethod=RotationSequence  FollAlignAxisA=+X  BaseAlignAxisA=+Y  FollAlignAxisB=+Y  BaseAlignAxisB=+Z  RotationStandardAxis=+Z  RotationAngle=0  RotationAngleUnits=deg  RotationArbitraryAxis=[0 0 1]  RotationSequenceAxes=BaseAxes  RotationSequence=XYZ  RotationSequenceAngles=[0, -0, 0]  RotationSequenceAnglesUnits=rad  RotationMatrix=[1 0 0;0 1 0;0 0 1]  Quaternion=[1 0 0 0]  TranslationMethod=Cartesian  TranslationCartesianOffset=[0, 0, 0]  TranslationCartesianOffsetUnits=m  TranslationStandardAxis=+Z  TranslationStandardOffset=0  TranslationStandardOffsetUnits=m  TranslationROffset=0  TranslationROffsetUnits=m  TranslationThetaOffset=0  TranslationThetaOffsetUnits=deg  TranslationZOffset=0  TranslationZOffsetUnits=m
  F : PMIOPort  Side=Left
  F2 : PMIOPort  Port=2  Side=Right
  F1 : PMIOPort  Port=3  Side=Right
  connections:
  base_link_base_OriginTransform/LConn1 -- ReferenceFrame/RConn1 -- joint_1_OriginTransform/LConn1 -- F/RConn1 -- Visual/RConn1
  base_link_base_OriginTransform/RConn1 -- F1/RConn1
  joint_1_AxisTransform/RConn1 -- F2/RConn1
  joint_1_AxisTransform/LConn1 -- joint_1_OriginTransform/RConn1

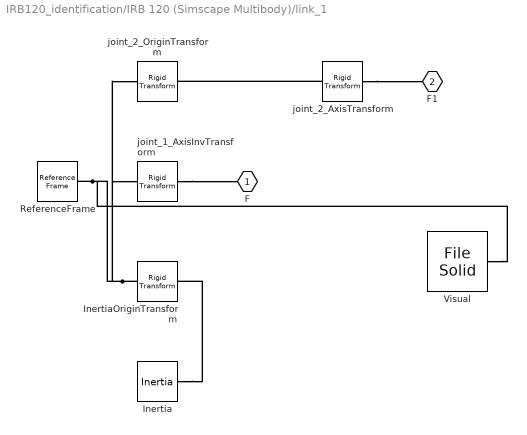
== system IRB120_identification/IRB 120 (Simscape Multibody)/link_1 ==
  Inertia : sm_lib/Body Elements/Inertia  InertiaType=Custom  Mass=3.067  MassUnits=kg  CenterOfMass=[0, 0, 0]  CenterOfMassUnits=m  MomentsOfInertia=[0.01421749999999999, 0.0144041, 0.0104533]  MomentsOfInertiaUnits=kg*m^2  ProductsOfInertia=[1.93404e-05, -2.31364e-05, -1.28579e-05]  ProductsOfInertiaUnits=kg*m^2  GraphicType=None  MarkerShape=Inertia  MarkerSize=20  GraphicVisPropType=SimpleVisualProperties  GraphicDiffuseColor=[0.5 0.5 0.5]  GraphicOpacity=1  GraphicSpecularColor=[0.5 0.5 0.5 1.0]  GraphicAmbientColor=[0.15 0.15 0.15 1.0]  GraphicEmissiveColor=[0.0 0.0 0.0 1.0]  GraphicShininess=75
  InertiaOriginTransform : sm_lib/Frames and Transforms/Rigid Transform  RotationMethod=RotationSequence  FollAlignAxisA=+X  BaseAlignAxisA=+Y  FollAlignAxisB=+Y  BaseAlignAxisB=+Z  RotationStandardAxis=+Z  RotationAngle=0  RotationAngleUnits=deg  RotationArbitraryAxis=[0 0 1]  RotationSequenceAxes=BaseAxes  RotationSequence=XYZ  RotationSequenceAngles=[0, 0, 0]  RotationSequenceAnglesUnits=rad  RotationMatrix=[1 0 0;0 1 0;0 0 1]  Quaternion=[1 0 0 0]  TranslationMethod=Cartesian  TranslationCartesianOffset=[9.77e-05, -0.00012, 0.23841]  TranslationCartesianOffsetUnits=m  TranslationStandardAxis=+Z  TranslationStandardOffset=0  TranslationStandardOffsetUnits=m  TranslationROffset=0  TranslationROffsetUnits=m  TranslationThetaOffset=0  TranslationThetaOffsetUnits=deg  TranslationZOffset=0  TranslationZOffsetUnits=m
  ReferenceFrame : sm_lib/Frames and Transforms/Reference Frame
  Visual : sm_lib/Body Elements/File Solid  ExtGeomFileName=IRB120_link_1.stl  UnitType=Custom  ExtGeomFileUnits=m  StepReaderType=HEX  ExportConvexHullGeometry=off  InertiaType=PointMass  BasedOnType=DensityFromFile  Density=1000  DensityUnits=kg/m^3  Mass=0  MassUnits=kg  CenterOfMass=[0 0 0]  CenterOfMassUnits=m  MomentsOfInertia=[1 1 1]  MomentsOfInertiaUnits=kg*m^2  ProductsOfInertia=[0 0 0]  ProductsOfInertiaUnits=kg*m^2  GraphicType=FromGeometry  MarkerShape=Sphere  MarkerSize=10  GraphicVisPropType=SimpleVisualProperties  GraphicDiffuseColor=[0.95 0.55 0.22]  GraphicOpacity=1  GraphicSpecularColor=[0.5 0.5 0.5 1.0]  GraphicAmbientColor=[0.15 0.15 0.15 1.0]  GraphicEmissiveColor=[0.0 0.0 0.0 1.0]  GraphicShininess=75  DoExposeReferenceFrame=on  SerializedFrames=<Frames/>
  joint_1_AxisInvTransform : sm_lib/Frames and Transforms/Rigid Transform  RotationMethod=ArbitraryAxis  FollAlignAxisA=+X  BaseAlignAxisA=+Y  FollAlignAxisB=+Y  BaseAlignAxisB=+Z  RotationStandardAxis=+Z  RotationAngle=0  RotationAngleUnits=rad  RotationArbitraryAxis=[1, 0, 0]  RotationSequenceAxes=FollowerAxes  RotationSequence=XYX  RotationSequenceAngles=[0 0 0]  RotationSequenceAnglesUnits=deg  RotationMatrix=[1 0 0;0 1 0;0 0 1]  Quaternion=[1 0 0 0]  TranslationMethod=Cartesian  TranslationCartesianOffset=[0, 0, 0]  TranslationCartesianOffsetUnits=m  TranslationStandardAxis=+Z  TranslationStandardOffset=0  TranslationStandardOffsetUnits=m  TranslationROffset=0  TranslationROffsetUnits=m  TranslationThetaOffset=0  TranslationThetaOffsetUnits=deg  TranslationZOffset=0  TranslationZOffsetUnits=m
  joint_2_AxisTransform : sm_lib/Frames and Transforms/Rigid Transform  RotationMethod=ArbitraryAxis  FollAlignAxisA=+X  BaseAlignAxisA=+Y  FollAlignAxisB=+Y  BaseAlignAxisB=+Z  RotationStandardAxis=+Z  RotationAngle=1.570796326794897  RotationAngleUnits=rad  RotationArbitraryAxis=[-1, 0, 0]  RotationSequenceAxes=FollowerAxes  RotationSequence=XYX  RotationSequenceAngles=[0 0 0]  RotationSequenceAnglesUnits=deg  RotationMatrix=[1 0 0;0 1 0;0 0 1]  Quaternion=[1 0 0 0]  TranslationMethod=Cartesian  TranslationCartesianOffset=[0, 0, 0]  TranslationCartesianOffsetUnits=m  TranslationStandardAxis=+Z  TranslationStandardOffset=0  TranslationStandardOffsetUnits=m  TranslationROffset=0  TranslationROffsetUnits=m  TranslationThetaOffset=0  TranslationThetaOffsetUnits=deg  TranslationZOffset=0  TranslationZOffsetUnits=m
  joint_2_OriginTransform : sm_lib/Frames and Transforms/Rigid Transform  RotationMethod=RotationSequence  FollAlignAxisA=+X  BaseAlignAxisA=+Y  FollAlignAxisB=+Y  BaseAlignAxisB=+Z  RotationStandardAxis=+Z  RotationAngle=0  RotationAngleUnits=deg  RotationArbitraryAxis=[0 0 1]  RotationSequenceAxes=BaseAxes  RotationSequence=XYZ  RotationSequenceAngles=[0, -0, 0]  RotationSequenceAnglesUnits=rad  RotationMatrix=[1 0 0;0 1 0;0 0 1]  Quaternion=[1 0 0 0]  TranslationMethod=Cartesian  TranslationCartesianOffset=[0, 0, 0.29]  TranslationCartesianOffsetUnits=m  TranslationStandardAxis=+Z  TranslationStandardOffset=0  TranslationStandardOffsetUnits=m  TranslationROffset=0  TranslationROffsetUnits=m  TranslationThetaOffset=0  TranslationThetaOffsetUnits=deg  TranslationZOffset=0  TranslationZOffsetUnits=m
  F : PMIOPort  Side=Left
  F1 : PMIOPort  Port=2  Side=Right
  connections:
  Inertia/RConn1 -- InertiaOriginTransform/RConn1
  InertiaOriginTransform/LConn1 -- joint_1_AxisInvTransform/LConn1 -- joint_2_OriginTransform/LConn1 -- ReferenceFrame/RConn1 -- Visual/RConn1
  joint_1_AxisInvTransform/RConn1 -- F/RConn1
  joint_2_AxisTransform/RConn1 -- F1/RConn1
  joint_2_AxisTransform/LConn1 -- joint_2_OriginTransform/RConn1

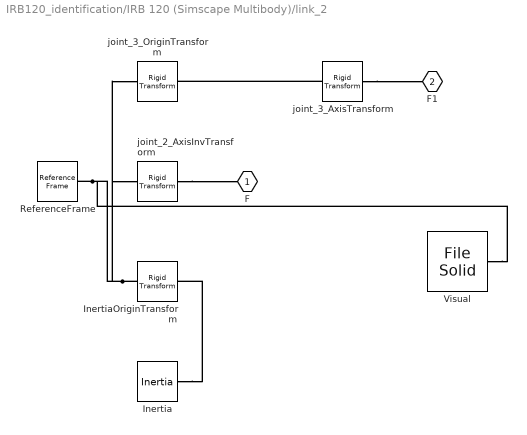
== system IRB120_identification/IRB 120 (Simscape Multibody)/link_2 ==
  Inertia : sm_lib/Body Elements/Inertia  InertiaType=Custom  Mass=3.909  MassUnits=kg  CenterOfMass=[0, 0, 0]  CenterOfMassUnits=m  MomentsOfInertia=[0.06031110000000001, 0.04156900000000001, 0.0259548]  MomentsOfInertiaUnits=kg*m^2  ProductsOfInertia=[-0.00050497, 5.724069999999998e-05, 9.834310000000001e-06]  ProductsOfInertiaUnits=kg*m^2  GraphicType=None  MarkerShape=Inertia  MarkerSize=20  GraphicVisPropType=SimpleVisualProperties  GraphicDiffuseColor=[0.5 0.5 0.5]  GraphicOpacity=1  GraphicSpecularColor=[0.5 0.5 0.5 1.0]  GraphicAmbientColor=[0.15 0.15 0.15 1.0]  GraphicEmissiveColor=[0.0 0.0 0.0 1.0]  GraphicShininess=75
  InertiaOriginTransform : sm_lib/Frames and Transforms/Rigid Transform  RotationMethod=RotationSequence  FollAlignAxisA=+X  BaseAlignAxisA=+Y  FollAlignAxisB=+Y  BaseAlignAxisB=+Z  RotationStandardAxis=+Z  RotationAngle=0  RotationAngleUnits=deg  RotationArbitraryAxis=[0 0 1]  RotationSequenceAxes=BaseAxes  RotationSequence=XYZ  RotationSequenceAngles=[0, 0, 0]  RotationSequenceAnglesUnits=rad  RotationMatrix=[1 0 0;0 1 0;0 0 1]  Quaternion=[1 0 0 0]  TranslationMethod=Cartesian  TranslationCartesianOffset=[0.00078, -0.00212, 0.10124]  TranslationCartesianOffsetUnits=m  TranslationStandardAxis=+Z  TranslationStandardOffset=0  TranslationStandardOffsetUnits=m  TranslationROffset=0  TranslationROffsetUnits=m  TranslationThetaOffset=0  TranslationThetaOffsetUnits=deg  TranslationZOffset=0  TranslationZOffsetUnits=m
  ReferenceFrame : sm_lib/Frames and Transforms/Reference Frame
  Visual : sm_lib/Body Elements/File Solid  ExtGeomFileName=IRB120_link_2.stl  UnitType=Custom  ExtGeomFileUnits=m  StepReaderType=HEX  ExportConvexHullGeometry=off  InertiaType=PointMass  BasedOnType=DensityFromFile  Density=1000  DensityUnits=kg/m^3  Mass=0  MassUnits=kg  CenterOfMass=[0 0 0]  CenterOfMassUnits=m  MomentsOfInertia=[1 1 1]  MomentsOfInertiaUnits=kg*m^2  ProductsOfInertia=[0 0 0]  ProductsOfInertiaUnits=kg*m^2  GraphicType=FromGeometry  MarkerShape=Sphere  MarkerSize=10  GraphicVisPropType=SimpleVisualProperties  GraphicDiffuseColor=[0.18 0.53 0.76]  GraphicOpacity=1  GraphicSpecularColor=[0.5 0.5 0.5 1.0]  GraphicAmbientColor=[0.15 0.15 0.15 1.0]  GraphicEmissiveColor=[0.0 0.0 0.0 1.0]  GraphicShininess=75  DoExposeReferenceFrame=on  SerializedFrames=<Frames/>
  joint_2_AxisInvTransform : sm_lib/Frames and Transforms/Rigid Transform  RotationMethod=ArbitraryAxis  FollAlignAxisA=+X  BaseAlignAxisA=+Y  FollAlignAxisB=+Y  BaseAlignAxisB=+Z  RotationStandardAxis=+Z  RotationAngle=1.570796326794897  RotationAngleUnits=rad  RotationArbitraryAxis=[-1, 0, 0]  RotationSequenceAxes=FollowerAxes  RotationSequence=XYX  RotationSequenceAngles=[0 0 0]  RotationSequenceAnglesUnits=deg  RotationMatrix=[1 0 0;0 1 0;0 0 1]  Quaternion=[1 0 0 0]  TranslationMethod=Cartesian  TranslationCartesianOffset=[0, 0, 0]  TranslationCartesianOffsetUnits=m  TranslationStandardAxis=+Z  TranslationStandardOffset=0  TranslationStandardOffsetUnits=m  TranslationROffset=0  TranslationROffsetUnits=m  TranslationThetaOffset=0  TranslationThetaOffsetUnits=deg  TranslationZOffset=0  TranslationZOffsetUnits=m
  joint_3_AxisTransform : sm_lib/Frames and Transforms/Rigid Transform  RotationMethod=ArbitraryAxis  FollAlignAxisA=+X  BaseAlignAxisA=+Y  FollAlignAxisB=+Y  BaseAlignAxisB=+Z  RotationStandardAxis=+Z  RotationAngle=1.570796326794897  RotationAngleUnits=rad  RotationArbitraryAxis=[-1, 0, 0]  RotationSequenceAxes=FollowerAxes  RotationSequence=XYX  RotationSequenceAngles=[0 0 0]  RotationSequenceAnglesUnits=deg  RotationMatrix=[1 0 0;0 1 0;0 0 1]  Quaternion=[1 0 0 0]  TranslationMethod=Cartesian  TranslationCartesianOffset=[0, 0, 0]  TranslationCartesianOffsetUnits=m  TranslationStandardAxis=+Z  TranslationStandardOffset=0  TranslationStandardOffsetUnits=m  TranslationROffset=0  TranslationROffsetUnits=m  TranslationThetaOffset=0  TranslationThetaOffsetUnits=deg  TranslationZOffset=0  TranslationZOffsetUnits=m
  joint_3_OriginTransform : sm_lib/Frames and Transforms/Rigid Transform  RotationMethod=RotationSequence  FollAlignAxisA=+X  BaseAlignAxisA=+Y  FollAlignAxisB=+Y  BaseAlignAxisB=+Z  RotationStandardAxis=+Z  RotationAngle=0  RotationAngleUnits=deg  RotationArbitraryAxis=[0 0 1]  RotationSequenceAxes=BaseAxes  RotationSequence=XYZ  RotationSequenceAngles=[0, -0, 0]  RotationSequenceAnglesUnits=rad  RotationMatrix=[1 0 0;0 1 0;0 0 1]  Quaternion=[1 0 0 0]  TranslationMethod=Cartesian  TranslationCartesianOffset=[0, 0, 0.27]  TranslationCartesianOffsetUnits=m  TranslationStandardAxis=+Z  TranslationStandardOffset=0  TranslationStandardOffsetUnits=m  TranslationROffset=0  TranslationROffsetUnits=m  TranslationThetaOffset=0  TranslationThetaOffsetUnits=deg  TranslationZOffset=0  TranslationZOffsetUnits=m
  F : PMIOPort  Side=Left
  F1 : PMIOPort  Port=2  Side=Right
  connections:
  Inertia/RConn1 -- InertiaOriginTransform/RConn1
  InertiaOriginTransform/LConn1 -- joint_2_AxisInvTransform/LConn1 -- joint_3_OriginTransform/LConn1 -- ReferenceFrame/RConn1 -- Visual/RConn1
  joint_2_AxisInvTransform/RConn1 -- F/RConn1
  joint_3_AxisTransform/RConn1 -- F1/RConn1
  joint_3_AxisTransform/LConn1 -- joint_3_OriginTransform/RConn1
